simulink model "Matlab_Controller_UCS"  (R2026a)
settings: Solver=FixedStepDiscrete  StopTime=S.tspan  FixedStep=S.dt_sim  RelTol=rel_tol  AbsTol=abs_tol
undefined symbols (not defined in the file): I, P, S
libraries: simulink x1, mspsensorlib x1
PreSaveFcn:
  | defaultToFileBlockNames(bdroot);
settings Model: Creator=koryh  LastModifiedBy=kjhaydon
settings SimscapeCC: SimscapeNominalValues="[{\"value\":\"1\",\"unit\":\"A\"},{\"value\":\"1\",\"unit\":\"bar\"},{\"value\":\"1\",\"unit\":\"cm^2\"},{\"value\":\"1\",\"unit\":\"cm^3/s\"},{\"value\":\"1\",\"unit\":\"kJ/kg\"},{\"value\":\"1\",\"unit\":\"kW\"},{\"value\":\"1\",\"unit\":\"l\"},{\"value\":\"1\",\"unit\":\"N\"},{\"value\":\"1\",\"unit\":\"N*m\"},{\"value\":\"1\",\"unit\":\"V\"}]"  SimscapeLogType=none  SimscapeLogDataHistory=5000.0

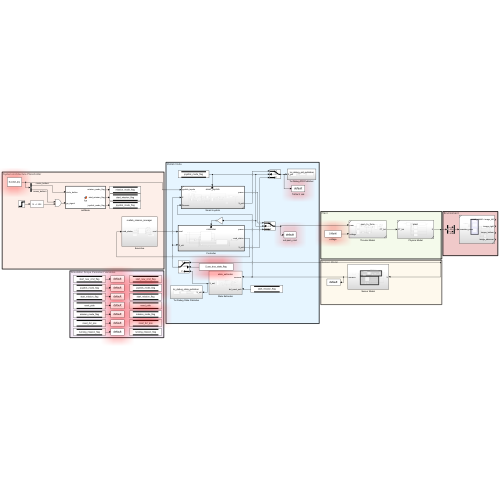
[thumbnail: Simulink's stored preview of the top-level diagram]
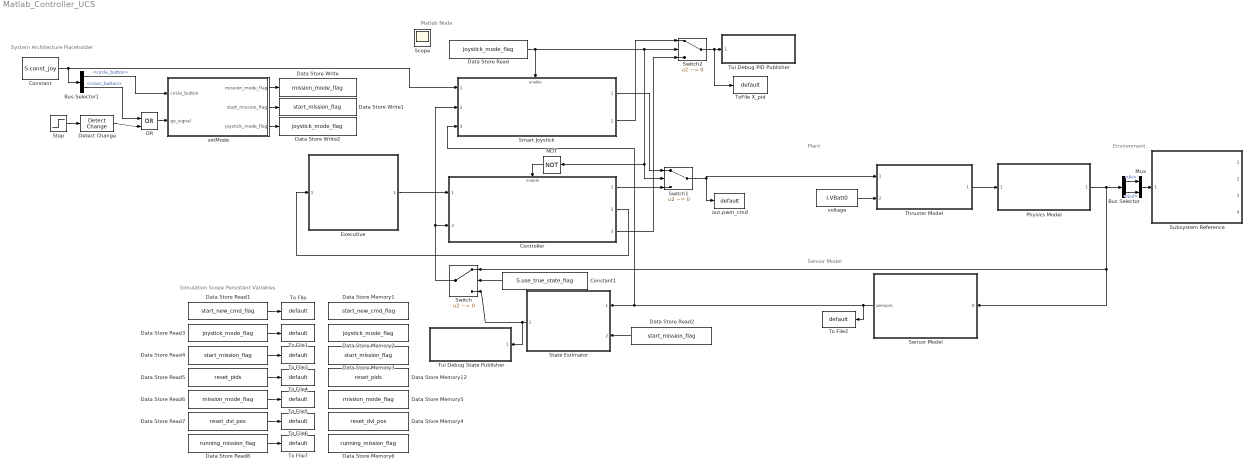
== system Matlab_Controller_UCS ==
  note: Environment
  note: System Architecture Placeholder
  note: Sensor Model
  note: Simulation Scope Persistant Variables
  note: Plant
  note: Matlab Node
  Bus Selector : BusSelector  OutputSignals=Ri,Eul
  Bus Selector1 : BusSelector  OutputSignals=circle_button,cross_button
  Constant : Constant  Value=S.const_joy  OutDataTypeStr=Bus: joystick_bus
  Constant1 : Constant  Value=S.use_true_state_flag
  Controller : Subsystem  ReferencedSubsystem=controller
  Data Store Memory1 : DataStoreMemory  DataStoreName=start_new_cmd_flag  WriteAfterWriteMsg=warning  InitialValue=true  ShowAdditionalParam=off  OutDataTypeStr=boolean
  Data Store Memory12 : DataStoreMemory  DataStoreName=reset_pids  WriteAfterWriteMsg=warning  InitialValue=false  ShowAdditionalParam=off  OutDataTypeStr=boolean
  Data Store Memory2 : DataStoreMemory  DataStoreName=joystick_mode_flag  WriteAfterWriteMsg=warning  InitialValue=S.initial_joystick_mode_enabled_flag  ShowAdditionalParam=off  OutDataTypeStr=boolean
  Data Store Memory3 : DataStoreMemory  DataStoreName=start_mission_flag  WriteAfterWriteMsg=warning  InitialValue=false  ShowAdditionalParam=off  OutDataTypeStr=boolean
  Data Store Memory4 : DataStoreMemory  DataStoreName=reset_dvl_pos  WriteAfterWriteMsg=warning  InitialValue=false  ShowAdditionalParam=off  OutDataTypeStr=boolean
  Data Store Memory5 : DataStoreMemory  DataStoreName=mission_mode_flag  WriteAfterWriteMsg=warning  InitialValue=~S.initial_joystick_mode_enabled_flag  ShowAdditionalParam=off  OutDataTypeStr=boolean
  Data Store Memory6 : DataStoreMemory  DataStoreName=running_mission_flag  WriteAfterWriteMsg=warning  InitialValue=false  ShowAdditionalParam=off  OutDataTypeStr=boolean
  Data Store Read : DataStoreRead  DataStoreName=joystick_mode_flag  IndexOptions=Index vector (dialog)  Indices=1  OutputSizes=1
  Data Store Read1 : DataStoreRead  DataStoreName=start_new_cmd_flag  IndexOptions=Index vector (dialog)  Indices=1  OutputSizes=1
  Data Store Read2 : DataStoreRead  DataStoreName=start_mission_flag  IndexOptions=Index vector (dialog)  Indices=1  OutputSizes=1
  Data Store Read3 : DataStoreRead  DataStoreName=joystick_mode_flag  IndexOptions=Index vector (dialog)  Indices=1  OutputSizes=1
  Data Store Read4 : DataStoreRead  DataStoreName=start_mission_flag  IndexOptions=Index vector (dialog)  Indices=1  OutputSizes=1
  Data Store Read5 : DataStoreRead  DataStoreName=reset_pids  IndexOptions=Index vector (dialog)  Indices=1  OutputSizes=1
  Data Store Read6 : DataStoreRead  DataStoreName=mission_mode_flag  IndexOptions=Index vector (dialog)  Indices=1  OutputSizes=1
  Data Store Read7 : DataStoreRead  DataStoreName=reset_dvl_pos  IndexOptions=Index vector (dialog)  Indices=1  OutputSizes=1
  Data Store Read8 : DataStoreRead  DataStoreName=running_mission_flag  IndexOptions=Index vector (dialog)  Indices=1  OutputSizes=1
  Data Store Write : DataStoreWrite  DataStoreName=mission_mode_flag  IndexOptions=Index vector (dialog)  Indices=1  OutputSizes=1
  Data Store Write1 : DataStoreWrite  DataStoreName=start_mission_flag  IndexOptions=Index vector (dialog)  Indices=1  OutputSizes=1
  Data Store Write2 : DataStoreWrite  DataStoreName=joystick_mode_flag  IndexOptions=Index vector (dialog)  Indices=1  OutputSizes=1
  Detect Change : simulink/Logic and Bit Operations/Detect Change  vinit=0  OutDataTypeStr=boolean
  Executive : Subsystem  ReferencedSubsystem=matlab_mission_manager
  Mux : Mux  Inputs=2
  NOT : Logic  Operator=NOT  IconShape=distinctive  AllPortsSameDT=off  OutDataTypeStr=boolean
  OR : Logic  Operator=OR  IconShape=distinctive  AllPortsSameDT=off  OutDataTypeStr=boolean
  Physics Model : Subsystem  ReferencedSubsystem=plant
  Sensor Model : Subsystem
  Smart Joystick : Subsystem  ReferencedSubsystem=smart_joystick
  State Estimator : Subsystem  ReferencedSubsystem=state_estimator
  Step : Step  SampleTime=0
  Subsystem Reference : Subsystem  ReferencedSubsystem=unreal_cosim
  Switch : Switch  Criteria=u2 ~= 0  SaturateOnIntegerOverflow=off  InputSameDT=off
  Switch1 : Switch  Criteria=u2 ~= 0  SaturateOnIntegerOverflow=off  InputSameDT=off
  Switch2 : Switch  Criteria=u2 ~= 0  SaturateOnIntegerOverflow=off  InputSameDT=off
  Thruster Model : Subsystem  ReferencedSubsystem=pwm_to_force
  To File : ToFile  Filename=default  MatrixName=start_new_cmd_flag  SaveFormat=Timeseries  SampleTime=S.dt_control
  To File1 : ToFile  Filename=default  MatrixName=joystick_mode_flag  SaveFormat=Timeseries  SampleTime=S.dt_control
  To File2 : ToFile  Filename=default  MatrixName=sensors  SaveFormat=Timeseries
  To File3 : ToFile  Filename=default  MatrixName=start_mission_flag  SaveFormat=Timeseries  SampleTime=S.dt_control
  To File4 : ToFile  Filename=default  MatrixName=reset_pids  SaveFormat=Timeseries  SampleTime=S.dt_control
  To File5 : ToFile  Filename=default  MatrixName=mission_mode_flag  SaveFormat=Timeseries  SampleTime=S.dt_control
  To File6 : ToFile  Filename=default  MatrixName=reset_dvl_pos  SaveFormat=Timeseries  SampleTime=S.dt_control
  To File7 : ToFile  Filename=default  MatrixName=running_mission_flag  SaveFormat=Timeseries  SampleTime=S.dt_control
  ToFile X_pid : ToFile  Filename=default  MatrixName=X_pid  SaveFormat=Timeseries  SampleTime=S.dt_data
  Tui Debug PID Publisher : Subsystem  ReferencedSubsystem=tui_debug_pid_publisher
  Tui Debug State Publisher : Subsystem  ReferencedSubsystem=tui_debug_state_publisher
  out.pwm_cmd : ToFile  Filename=default  MatrixName=pwm_ctrl  SaveFormat=Timeseries  SampleTime=S.dt_data
  setMode : MATLAB Function  TreatAsAtomicUnit=on
  voltage : Constant  Value=I.VBatt0
  Scope : Scope
      settings: ActiveDisplayYMinimum=-0.048832566475369238  ActiveDisplayYMaximum=0.79721663606048965
  wires:
  Bus Selector/2 -> Mux/2  "<Eul>"
  Mux/1 -> Subsystem Reference/1
  Bus Selector/1 -> Mux/1  "<Ri>"
  Smart Joystick/2 -> Switch2/1
  Data Store Read6/1 -> To File5/1
  Controller/3 -> Switch2/3
  Data Store Read5/1 -> To File4/1
  Smart Joystick/1 -> Switch1/1
  State Estimator/1 -> Switch/3, Tui Debug State Publisher/1
  Bus Selector1/1 -> setMode/1(circle_button)  "<circle_button>"
  Switch/1 -> Smart Joystick/2, Controller/2
  Executive/1 -> Controller/1
  Step/1 -> Detect Change/1
  setMode/1(mission_mode_flag) -> Data Store Write/1
  Controller/2 -> Executive/1
  Physics Model/1 -> Bus Selector/1, Switch/1, Sensor Model/1(X)
  Data Store Read2/1 -> State Estimator/2
  setMode/3(joystick_mode_flag) -> Data Store Write2/1
  voltage/1 -> Thruster Model/2
  Detect Change/1 -> OR/2
  Data Store Read4/1 -> To File3/1
  Thruster Model/1 -> Physics Model/1
  Data Store Read8/1 -> To File7/1
  OR/1 -> setMode/2(go_signal)
  Data Store Read3/1 -> To File1/1
  Switch1/1 -> out.pwm_cmd/1, Thruster Model/1
  Data Store Read/1 -> Switch1/2, NOT/1, Switch2/2, Smart Joystick/Enable
  NOT/1 -> Controller/Enable
  setMode/2(start_mission_flag) -> Data Store Write1/1
  Switch2/1 -> ToFile X_pid/1, Tui Debug PID Publisher/1
  Bus Selector1/2 -> OR/1  "<cross_button>"
  Data Store Read7/1 -> To File6/1
  Sensor Model/1(sensors) -> To File2/1, State Estimator/1, Smart Joystick/3
  Data Store Read1/1 -> To File/1
  Constant1/1 -> Switch/2
  Constant/1 -> Bus Selector1/1, Smart Joystick/1
  Controller/1 -> Switch1/3

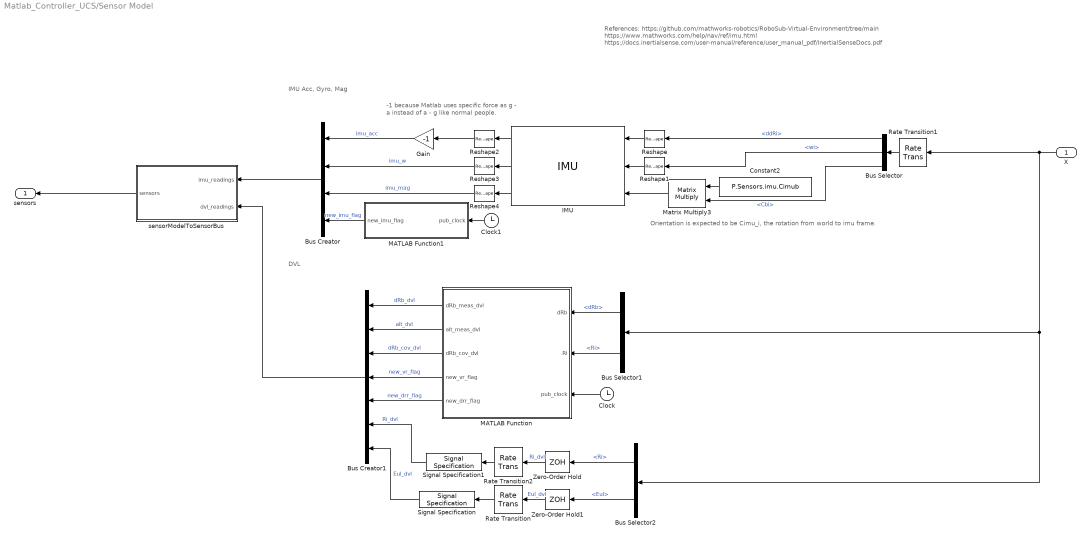
== system Matlab_Controller_UCS/Sensor Model ==
  note: IMU Acc, Gyro, Mag
  note: -1 because Matlab uses specific force as
      |  g - a instead of a - g like normal people.
  note: Orientation is expected to be Cimu_i, the rotation from world to imu frame.
  note: References:
      | https://github.com/mathworks-robotics/RoboSub-Virtual-Environment/tree/main
      | https://www.mathworks.com/help/nav/ref/imu.html
      | https://docs.inertialsense.com/user-manual/reference/user_manual_pdf/InertialSenseDocs.pdf
  note: DVL
  X : Inport  OutDataTypeStr=Bus: X_bus  SampleTime=S.dt_control
  Bus Creator : BusCreator  Inputs=4  OutDataTypeStr=Bus: imu_bus
  Bus Creator1 : BusCreator  Inputs=7  OutDataTypeStr=Bus: dvl_bus
  Bus Selector : BusSelector  OutputSignals=ddRi,wi,Cbi
  Bus Selector1 : BusSelector  OutputSignals=dRb,Ri
  Bus Selector2 : BusSelector  OutputSignals=Ri,Eul
  Clock : Clock
  Clock1 : Clock
  Constant2 : Constant  Value=P.Sensors.imu.Cimub
  Gain : Gain  Gain=-1
  IMU : mspsensorlib/IMU  DispRefFrame=NED  TemperaturePort=off  Temperature=P.Sensors.imu.T  MagneticFieldPort=off  MagneticFieldNED=P.Sensors.imu.Bi  MagneticFieldENU=[ -2.4169, 27.5550, 16.0849 ]  SeedDouble=67  SimulateUsing=Interpreted execution  AccelParamsMeasurementRange=P.Sensors.imu.acc.meas_range  AccelParamsResolution=P.Sensors.imu.acc.res  AccelParamsConstantBias=P.Sensors.imu.acc.const_bias  AccelParamsAxesMisalignment=P.Sensors.imu.acc.axes_skew  AccelParamsNoiseDensity=P.Sensors.imu.acc.vel_rand_walk  AccelParamsBiasInstability=P.Sensors.imu.acc.bias_inst  AccelParamsBiasInstabilityNumerator=P.Sensors.imu.acc.bias_inst_num_coeffs  AccelParamsBiasInstabilityDenominator=P.Sensors.imu.acc.bias_inst_den_coeffs  AccelParamsRandomWalk=P.Sensors.imu.acc.acc_rand_walk  AccelParamsNoiseType=double-sided  AccelParamsTemperatureBias=P.Sensors.imu.acc.temp_bias  AccelParamsTemperatureScaleFactor=P.Sensors.imu.acc.temp_scale_factor  GyroParamsMeasurementRange=P.Sensors.imu.gyro.max_read  GyroParamsResolution=P.Sensors.imu.gyro.res  GyroParamsConstantBias=P.Sensors.imu.gyro.const_bias  GyroParamsAxesMisalignment=P.Sensors.imu.gyro.axes_skew  GyroParamsAccelerationBias=P.Sensors.imu.gyro.bias_from_acc  GyroParamsNoiseDensity=P.Sensors.imu.gyro.angle_rand_walk  GyroParamsBiasInstability=P.Sensors.imu.gyro.bias_inst  GyroParamsBiasInstabilityNumerator=P.Sensors.imu.gyro.bias_inst_filter_num_coeffs  GyroParamsBiasInstabilityDenominator=P.Sensors.imu.gyro.bias_inst_filter_den_coeffs  GyroParamsRandomWalk=P.Sensors.imu.gyro.rate_rand_walk  GyroParamsNoiseType=double-sided  GyroParamsTemperatureBias=P.Sensors.imu.gyro.temp_bias  GyroParamsTemperatureScaleFactor=P.Sensors.imu.gyro.temp_scale_factor  MagParamsMeasurementRange=P.Sensors.imu.mag.max_read  MagParamsResolution=P.Sensors.imu.mag.res  MagParamsConstantBias=P.Sensors.imu.mag.const_bias  MagParamsAxesMisalignment=P.Sensors.imu.mag.axes_skew  MagParamsNoiseDensity=P.Sensors.imu.mag.white_noise_psd  MagParamsBiasInstability=P.Sensors.imu.mag.bias_inst  MagParamsBiasInstabilityNumerator=P.Sensors.imu.mag.bias_inst_filter_num_coeffs  MagParamsBiasInstabilityDenominator=P.Sensors.imu.mag.bias_isnt_filter_den_coeffs  MagParamsRandomWalk=P.Sensors.imu.mag.rand_walk  MagParamsNoiseType=double-sided  MagParamsTemperatureBias=P.Sensors.imu.mag.temp_bias  MagParamsTemperatureScaleFactor=P.Sensors.imu.mag.temp_scale_factor
  MATLAB Function : MATLAB Function  TreatAsAtomicUnit=on
  MATLAB Function1 : MATLAB Function  TreatAsAtomicUnit=on
  Matrix Multiply3 : Product  Multiplication=Matrix(*)
  Rate Transition : RateTransition  Deterministic=off  OutPortSampleTime=S.dt_control
  Rate Transition1 : RateTransition  OutPortSampleTime=S.dt_imu
  Rate Transition2 : RateTransition  Deterministic=off  OutPortSampleTime=S.dt_control
  Reshape : Reshape  OutputDimensionality=Row vector (2-D)
  Reshape1 : Reshape  OutputDimensionality=Row vector (2-D)
  Reshape2 : Reshape  OutputDimensionality=Column vector (2-D)
  Reshape3 : Reshape  OutputDimensionality=Column vector (2-D)
  Reshape4 : Reshape  OutputDimensionality=Column vector (2-D)
  Signal Specification : SignalSpecification  SampleTime=S.dt_control
  Signal Specification1 : SignalSpecification  SampleTime=S.dt_control
  Zero-Order Hold : ZeroOrderHold  SampleTime=S.dt_dvl_drr
  Zero-Order Hold1 : ZeroOrderHold  SampleTime=S.dt_dvl_drr
  sensorModelToSensorBus : MATLAB Function  TreatAsAtomicUnit=on
  sensors : Outport  OutDataTypeStr=Bus: sensor_bus  SampleTime=S.dt_control
  wires:
  X/1 -> Rate Transition1/1, Bus Selector2/1, Bus Selector1/1
  Reshape/1 -> IMU/1
  Bus Selector/2 -> Reshape1/1  "<wi>"
  IMU/1 -> Reshape2/1
  IMU/2 -> Reshape3/1
  IMU/3 -> Reshape4/1
  Reshape1/1 -> IMU/2
  Bus Selector/1 -> Reshape/1  "<ddRi>"
  Matrix Multiply3/1 -> IMU/3
  Constant2/1 -> Matrix Multiply3/1
  Bus Selector/3 -> Matrix Multiply3/2  "<Cbi>"
  Reshape2/1 -> Gain/1
  Bus Selector1/1 -> MATLAB Function/1(dRb)  "<dRb>"
  Bus Selector1/2 -> MATLAB Function/2(Ri)  "<Ri>"
  sensorModelToSensorBus/1(sensors) -> sensors/1
  Rate Transition1/1 -> Bus Selector/1
  Clock/1 -> MATLAB Function/3(pub_clock)
  Clock1/1 -> MATLAB Function1/1(pub_clock)
  Gain/1 -> Bus Creator/1  "imu_acc"
  Reshape3/1 -> Bus Creator/2  "imu_w"
  Reshape4/1 -> Bus Creator/3  "imu_mag"
  MATLAB Function1/1(new_imu_flag) -> Bus Creator/4  "new_imu_flag"
  MATLAB Function/1(dRb_meas_dvl) -> Bus Creator1/1  "dRb_dvl"
  MATLAB Function/2(alt_meas_dvl) -> Bus Creator1/2  "alt_dvl"
  MATLAB Function/3(dRb_cov_dvl) -> Bus Creator1/3  "dRb_cov_dvl"
  MATLAB Function/4(new_vr_flag) -> Bus Creator1/4  "new_vr_flag"
  MATLAB Function/5(new_drr_flag) -> Bus Creator1/5  "new_drr_flag"
  Bus Creator/1 -> sensorModelToSensorBus/1(imu_readings)
  Bus Creator1/1 -> sensorModelToSensorBus/2(dvl_readings)
  Zero-Order Hold/1 -> Rate Transition2/1  "Ri_dvl"
  Signal Specification1/1 -> Bus Creator1/6  "Ri_dvl"
  Signal Specification/1 -> Bus Creator1/7  "Eul_dvl"
  Rate Transition/1 -> Signal Specification/1
  Rate Transition2/1 -> Signal Specification1/1
  Zero-Order Hold1/1 -> Rate Transition/1  "Eul_dvl"
  Bus Selector2/1 -> Zero-Order Hold/1  "<Ri>"
  Bus Selector2/2 -> Zero-Order Hold1/1  "<Eul>"

== matlab function Matlab_Controller_UCS/Sensor Model/MATLAB Function1 ==
  settings: updateMethod=DISCRETE  sampleTime=S.dt_control
  data: pub_clock input; new_imu_flag output; S parameter
function new_imu_flag = fcn(pub_clock, S)

dt_imu = S.dt_imu;

persistent last_imu_time

if(isempty(last_imu_time))
    last_imu_time = pub_clock;
end


time_since_last_imu = pub_clock - last_imu_time;

if(time_since_last_imu < dt_imu)
    new_imu_flag = 0;
else
    new_imu_flag = 1;
    last_imu_time = pub_clock;
end

== matlab function Matlab_Controller_UCS/Sensor Model/MATLAB Function ==
  settings: updateMethod=DISCRETE  sampleTime=S.dt_control
  data: dRb input; dRb_meas_dvl output; Ri input; alt_meas_dvl output; dRb_cov_dvl output; pub_clock input; new_vr_flag output; new_drr_flag output; S parameter; P parameter
function [dRb_meas_dvl, alt_meas_dvl, dRb_cov_dvl, new_vr_flag, new_drr_flag] = dvl_sim(dRb, Ri, pub_clock, S, P)
%{
Model from this repository:
https://github.com/mathworks-robotics/RoboSub-Virtual-Environment/
Need to modify this to give erroneous or no reading when ground lock is
available.

Also need to add noise to the altitude measurement and determine if it
needs modification based on attitude.
%}

dt_dvl_vr = S.dt_dvl_vr;
dt_dvl_drr = S.dt_dvl_drr;

persistent last_drr_time
persistent last_vr_time

if(isempty(last_drr_time))
    last_drr_time = pub_clock;
end
if(isempty(last_vr_time))
    last_vr_time = pub_clock;
end

time_since_last_drr = pub_clock - last_drr_time;
time_since_last_vr = pub_clock - last_vr_time;
if(time_since_last_drr < dt_dvl_drr)
    new_drr_flag = 0;
else
    new_drr_flag = 1;
    last_drr_time = pub_clock;
end
if(time_since_last_vr < dt_dvl_vr)
    new_vr_flag = 0;
else
    new_vr_flag = 1;
    last_vr_time = pub_clock;
end



%get altitude (assumes Ri is measured from the robot's starting depth
true_depth = P.Sensors.dvl.start_depth + Ri(3); 
true_alt = P.Sensors.dvl.pool_depth - true_depth;
alt_meas_dvl = true_alt;

%bias for velocity measurements
persistent bias
if isempty(bias)
    bias = zeros(3,1);
end


% ---------------- Update bias (Gauss-Markov) ----------------
if P.Sensors.dvl.bias_tau > 0 && P.Sensors.dvl.bias_sigma_ss > 0
    % Discrete-time OU: b_{k+1} = (1 - dt/tau) b_k + sqrt(2*sigma^2*dt/tau) * w
    a = max(0.0, 1.0 - P.Sensors.dvl.bias_dt/P.Sensors.dvl.bias_tau);
    q = sqrt(max(0.0, 2.0*P.Sensors.dvl.bias_sigma_ss^2*P.Sensors.dvl.bias_dt/P.Sensors.dvl.bias_tau));
    bias = a*bias + q * randn(3,1);
else
    bias = zeros(3,1);
end

% ---------------- Add noise & bias ----------------
noise = P.Sensors.dvl.noise_sigma .* randn(3,1);    % white noise
dRb_meas_dvl = dRb + bias + noise;

dRb_cov_dvl = diag([P.Sensors.dvl.noise_sigma].^2);

== matlab function Matlab_Controller_UCS/Sensor Model/sensorModelToSensorBus ==
  settings: updateMethod=DISCRETE  sampleTime=S.dt_control
  data: imu_readings input; sensors output Bus: sensor_bus; dvl_readings input
function sensors = fcn(imu_readings, dvl_readings)

sensors = sensorModelToSensorBus(imu_readings, dvl_readings);

== matlab function Matlab_Controller_UCS/setMode ==
  data: circle_button input; go_signal input; mission_mode_flag output; start_mission_flag output; joystick_mode_flag output; S parameter
function [mission_mode_flag, start_mission_flag, joystick_mode_flag] = fcn(circle_button, go_signal, S)

persistent joystick_mode_flag_ mission_mode_flag_ 

%initial conditions set in createSim.m
if(isempty(joystick_mode_flag_))
    joystick_mode_flag_ = S.initial_joystick_mode_enabled_flag;
    mission_mode_flag_ = ~joystick_mode_flag_;
end

if(circle_button) %switch modes
    joystick_mode_flag_ = ~joystick_mode_flag_;
    mission_mode_flag_ = ~joystick_mode_flag_;
end

%send start signal
if(go_signal && joystick_mode_flag_)
    joystick_mode_flag_ = false;
    mission_mode_flag_ = true;
    start_mission_flag = true;
elseif(go_signal && mission_mode_flag_)
    joystick_mode_flag_ = false;
    mission_mode_flag_ = true;
    start_mission_flag = true;
else
    start_mission_flag = false;
end


mission_mode_flag = mission_mode_flag_;
joystick_mode_flag = joystick_mode_flag_;



end
